simulink model "Hinge"  (R2026b)
settings: Solver=VariableStepAuto
undefined symbols (not defined in the file): P, X, Y, Z
libraries: fl_lib x14, sm_lib x4
settings Model: Creator=amavromm  LastModifiedBy=amavromm

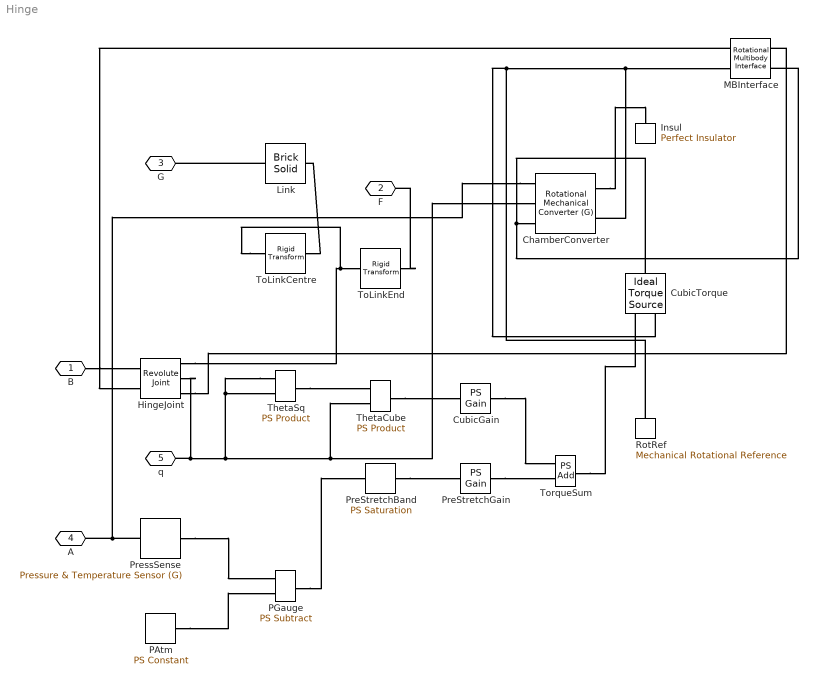
== system Hinge ==
  ChamberConverter : fl_lib/Gas/Elements/Rotational Mechanical Converter (G)  mech_orientation=foundation.enum.MechOrientationRotational.Positive  rotation_spec=foundation.enum.RotationSpec.InputSignal  theta_init=0 rad  volume_displacement=P.finger.D m^3/rad  dead_volume=P.finger.V0/P.finger.N_Joint m^3  area_A=P.gas.a_FingerPort m^2  environment_spec=foundation.enum.pressure_spec.atmospheric  environment_pressure=0.101325 MPa  p_I_specify=off  p_I_priority=High  p_I=P.gas.p_Init + P.gas.p_Atm Pa  p_I_nominal_specify=off  p_I_nominal_value=1  p_I_nominal_unit=MPa  T_I_specify=on  T_I_priority=High  T_I=P.gas.T_Amb K  T_I_nominal_specify=off  T_I_nominal_value=1  T_I_nominal_unit=K  rho_I_specify=off  rho_I_priority=None  rho_I=1.2 kg/m^3  rho_I_nominal_specify=off  rho_I_nominal_value=1  rho_I_nominal_unit=kg/m^3
  CubicGain : fl_lib/Physical Signals/Functions/PS Gain  gain=-P.finger.K3 N*m/rad^3
  CubicTorque : fl_lib/Mechanical/Mechanical Sources/Ideal Torque Source
  HingeJoint : sm_lib/Joints/Revolute Joint  JointMode=Normal  CompositeWrenchDir=FollowerOnBase  CompositeWrenchFrame=BaseFrame  SenseConstraintForce=off  SenseConstraintTorque=off  SenseTotalForce=off  SenseTotalTorque=off  PositionTargetSpecify=off  PositionTargetPriority=Low  PositionTargetValue=P.finger.theta_Init  PositionTargetValueUnits=rad  VelocityTargetSpecify=off  VelocityTargetPriority=High  VelocityTargetValue=0  VelocityTargetValueUnits=deg/s  EquilibriumPosition=0  EquilibriumPositionUnits=rad  SpringStiffness=P.finger.K  SpringStiffnessUnits=N*m/rad  DampingCoefficient=P.finger.c  DampingCoefficientUnits=N*m*s/rad  LowerLimitSpecify=off  LowerLimitBound=P.finger.theta_Min  LowerLimitBoundUnits=rad  LowerLimitStiffness=P.finger.k_Stop  LowerLimitStiffnessUnits=N*m/rad  LowerLimitDamping=P.finger.c  LowerLimitDampingUnits=N*m*s/rad  LowerLimitTransitionRegionWidth=P.finger.w_StopTrans  LowerLimitTransitionRegionWidthUnits=rad  UpperLimitSpecify=off  UpperLimitBound=90  UpperLimitBoundUnits=deg  UpperLimitStiffness=1e4  UpperLimitStiffnessUnits=N*m/deg  UpperLimitDamping=10  UpperLimitDampingUnits=N*m/(deg/s)  UpperLimitTransitionRegionWidth=0.1  UpperLimitTransitionRegionWidthUnits=deg  TorqueActuationMode=InputTorque  MotionActuationMode=ComputedMotion  SensePosition=on  SenseVelocity=on  SenseAcceleration=off  SenseTorqueForce=off  SenseLowerLimitTorqueForce=off  SenseUpperLimitTorqueForce=off
  Insul : fl_lib/Thermal/Thermal Elements/Perfect Insulator  T_specify=off  T_priority=None  T=293.15 K  T_nominal_specify=off  T_nominal_value=1  T_nominal_unit=K
  Link : sm_lib/Body Elements/Brick Solid  BrickDimensions=[P.finger.l_Link P.finger.h_Link P.finger.w_Link]  BrickDimensionsUnits=m  ExportEntireGeometry=on  InertiaType=CalculateFromGeometry  BasedOnType=Mass  Density=1000  DensityUnits=kg/m^3  Mass=P.finger.m_Link  MassUnits=kg  CenterOfMass=[0 0 0]  CenterOfMassUnits=m  MomentsOfInertia=[1 1 1]  MomentsOfInertiaUnits=kg*m^2  ProductsOfInertia=[0 0 0]  ProductsOfInertiaUnits=kg*m^2  GraphicType=FromGeometry  MarkerShape=Sphere  MarkerSize=10  GraphicVisPropType=SimpleVisualProperties  GraphicDiffuseColor=[0.96 0.58 0.22]  GraphicOpacity=1  GraphicSpecularColor=[0.5 0.5 0.5 1.0]  GraphicAmbientColor=[0.15 0.15 0.15 1.0]  GraphicEmissiveColor=[0.0 0.0 0.0 1.0]  GraphicShininess=75  DoExposeReferenceFrame=on  SerializedFrames=<Frames/>
  MBInterface : fl_lib/Mechanical/Multibody Interfaces/Rotational Multibody Interface
  PAtm : fl_lib/Physical Signals/Sources/PS Constant  constant=P.gas.p_Atm Pa
  PGauge : fl_lib/Physical Signals/Functions/PS Subtract
  PreStretchBand : fl_lib/Physical Signals/Nonlinear Operators/PS Saturation  upper_limit=P.finger.p0 Pa  lower_limit=0 Pa  ZeroCross=true
  PreStretchGain : fl_lib/Physical Signals/Functions/PS Gain  gain=-P.finger.D N*m/Pa
  PressSense : fl_lib/Gas/Sensors/Pressure & Temperature Sensor (G)  reference=foundation.enum.MeasurementReference.absolute  pressure=true  pressure_spec=foundation.enum.PressureMeasementSpec.Absolute  temperature=false
  RotRef : fl_lib/Mechanical/Rotational Elements/Mechanical Rotational Reference
  ThetaCube : fl_lib/Physical Signals/Functions/PS Product
  ThetaSq : fl_lib/Physical Signals/Functions/PS Product
  ToLinkCentre : sm_lib/Frames and Transforms/Rigid Transform  RotationMethod=None  FollAlignAxisA=+X  BaseAlignAxisA=+Y  FollAlignAxisB=+Y  BaseAlignAxisB=+Z  RotationStandardAxis=+Z  RotationAngle=0  RotationAngleUnits=deg  RotationArbitraryAxis=[0 0 1]  RotationSequenceAxes=FollowerAxes  RotationSequence=XYX  RotationSequenceAngles=[0 0 0]  RotationSequenceAnglesUnits=deg  RotationMatrix=[1 0 0;0 1 0;0 0 1]  Quaternion=[1 0 0 0]  TranslationMethod=Cartesian  TranslationCartesianOffset=[P.finger.l_Link/2 0 0]  TranslationCartesianOffsetUnits=m  TranslationStandardAxis=+Z  TranslationStandardOffset=0  TranslationStandardOffsetUnits=m  TranslationROffset=0  TranslationROffsetUnits=m  TranslationThetaOffset=0  TranslationThetaOffsetUnits=deg  TranslationZOffset=0  TranslationZOffsetUnits=m
  ToLinkEnd : sm_lib/Frames and Transforms/Rigid Transform  RotationMethod=None  FollAlignAxisA=+X  BaseAlignAxisA=+Y  FollAlignAxisB=+Y  BaseAlignAxisB=+Z  RotationStandardAxis=+Z  RotationAngle=0  RotationAngleUnits=deg  RotationArbitraryAxis=[0 0 1]  RotationSequenceAxes=FollowerAxes  RotationSequence=XYX  RotationSequenceAngles=[0 0 0]  RotationSequenceAnglesUnits=deg  RotationMatrix=[1 0 0;0 1 0;0 0 1]  Quaternion=[1 0 0 0]  TranslationMethod=Cartesian  TranslationCartesianOffset=[P.finger.l_Link 0 0]  TranslationCartesianOffsetUnits=m  TranslationStandardAxis=+Z  TranslationStandardOffset=0  TranslationStandardOffsetUnits=m  TranslationROffset=0  TranslationROffsetUnits=m  TranslationThetaOffset=0  TranslationThetaOffsetUnits=deg  TranslationZOffset=0  TranslationZOffsetUnits=m
  TorqueSum : fl_lib/Physical Signals/Functions/PS Add
  B : PMIOPort  Side=Left
  F : PMIOPort  Port=2  Side=Right
  G : PMIOPort  Port=3  Side=Right
  A : PMIOPort  Port=4  Side=Left
  q : PMIOPort  Port=5  Side=Right
  connections:
  Link/LConn1 -- G/RConn1
  ToLinkCentre/RConn1 -- Link/RConn1
  B/RConn1 -- HingeJoint/LConn1
  ToLinkCentre/LConn1 -- ToLinkEnd/LConn1 -- HingeJoint/RConn1
  ToLinkEnd/RConn1 -- F/RConn1
  MBInterface/LConn1 -- HingeJoint/LConn2
  HingeJoint/RConn3 -- MBInterface/RConn1
  ThetaSq/LConn1 -- ChamberConverter/LConn2 -- ThetaCube/LConn2 -- HingeJoint/RConn2 -- q/RConn1 -- ThetaSq/LConn2
  ThetaSq/RConn1 -- ThetaCube/LConn1
  ThetaCube/RConn1 -- CubicGain/LConn1
  ChamberConverter/LConn1 -- A/RConn1 -- PressSense/LConn1
  ChamberConverter/RConn1 -- Insul/LConn1
  MBInterface/RConn2 -- ChamberConverter/LConn3 -- CubicTorque/LConn1
  ChamberConverter/RConn2 -- RotRef/LConn1 -- CubicTorque/RConn2 -- MBInterface/LConn2
  PressSense/RConn1 -- PGauge/LConn1
  PAtm/RConn1 -- PGauge/LConn2
  PGauge/RConn1 -- PreStretchBand/LConn1
  PreStretchBand/RConn1 -- PreStretchGain/LConn1
  CubicGain/RConn1 -- TorqueSum/LConn1
  PreStretchGain/RConn1 -- TorqueSum/LConn2
  TorqueSum/RConn1 -- CubicTorque/RConn1
